simulink model "commhdlQPSKTxRx"  (R2025b)
settings: Solver=FixedStepDiscrete  StartTime=0.0  StopTime=stopTime  RelTol=1e-3
PostLoadFcn:
  | hScopeConfig = get_param([gcs '/Receiver/QPSK Rx/Frequency and Time Synchronizer/Symbol Synchronizer/No HDL/QPSK Receiver Eye Diagram'],'ScopeConfiguration');
  | 
  | hScopeConfig.OpenAtSimulationStart = false;
  | hScopeConfig.Visible = false;
  | SamplesPerSymbol = 4;
  | %UpsamplesRx = 1;
  | clear hScopeConfig
InitFcn:
  | commhdlQPSKTxRxModelInit;
  | % Rate bridge: ADRV9002/Jupiter radio runs at 15.36 MHz = 2x the 7.68 MHz
  | % (4 samples/symbol @ Rsym=1.92 MHz) the QPSK Rx requires. The deployed
  | % Receiver must downsample the ADC stream by 2. UpsamplesRx=1 fed the QPSK
  | % Rx 8 sps (2x-upsampled) and broke symbol sync / the loopback bit check.
  | UpsamplesRx = 1;   %% T8 RATE FIX: rail 15.36e6 == ADC bus rate,
  | %% no ingress decimation (was 2 when the rail sat on the 7.68e6 rung)
  | UpsamplesTx = 1;
  | clear simTimingOffset;
StopFcn:
  | if exist('simTimingOffset','var')
  |   disp('Simulation completed');
  |   %QPSKTxRxVerification;
  | end
undefined symbols (not defined in the file or in its folder): Add, Config, fsym, randsrc, RandStream, Rsym, Shift
libraries: hdlsllib x76, simulink x21, dspsigops x19, dsphdlfiltering2 x3, dsphdlsigops2 x2, dsphdlmathfun2 x2, commdigbbndpm3 x2, commchan3 x1, commrflib2 x1
(part 4 of 4)

== matlab function commhdlQPSKTxRx/Receiver/QPSK Rx/Frequency and Time Synchronizer/Packet Controller/sample discard controller ==
  data: dataIn input; validIn input; dataOut output; startIn input; endIn input; startOut output; endOut output; validOut output
function [dataOut,startOut,endOut,validOut] = controller(dataIn,validIn,startIn,endIn)
%#codegen

   persistent active dataOutReg validOutReg startOutReg endOutReg;
   if isempty(active)
      active  = false;
      dataOutReg = cast(0,'like',dataIn);
      validOutReg = false;
      startOutReg = false;
      endOutReg = false;
   end
   
   dataOut = dataOutReg;
   validOut = validOutReg;
   startOut = startOutReg;
   endOut = endOutReg;
   
   startOutReg = startIn;
   endOutReg = endIn;
   
   if startIn
       active = true;
   end
   
   if active
       dataOutReg(:) = dataIn;
       validOutReg = validIn;
   else
       dataOutReg(:) = 0;
       validOutReg = false;
   end
   
   if endIn
       if active 
           endOutReg = true;
       else
           endOutReg = false;
       end
       active = false;
   end
end

== matlab function commhdlQPSKTxRx/Receiver/QPSK Rx/Frequency and Time Synchronizer/Symbol Synchronizer/Interpolation Control ==
  data: mu output; Delta input; Underflow output
function [mu,Underflow] = Interpolation_ctrl(Delta)
% Implementation of modulo-1 counter for interpolation control listed in
% Figure 8.4.19 of "Digital Communications - A Discrete-Time Approach"
% by Michael Rice. See design details in Chapter 8.4.3 of the same book.
% 
% Input:
%   Delta - Loop filter output. If loop is in lock, delta would be small
% Output:
%   Underflow - Indicator of counter underflow. This is the strobe signal
%               for downstream processing
%   mu - Difference between actual sampling instant and the optimal instant,
%        between zero and one
%#codegen

% countReg - Counter value delayed by 1 sample
% muReg - The estimated timing error normalized by half QPSK symbols

   mask = fi(1-2^(-10),1,11,10);
   
   persistent countReg underflowReg muReg;
   if isempty(countReg)
       countReg  = fi(0,1,11,10);
       muReg = fi(0,1,11,10);
       underflowReg = false;
   end
   
   
   Underflow = underflowReg;
   mu = muReg;   
   
   
      % T8.4 anti-wedge clamp: if Delta <= -0.125 the decrementing counter
   % never underflows (strobes stop FOREVER -- Class-4 wedge / Class-1
   % episode mechanism; see tb_timing_wedge.v). Bound Delta so the
   % counter always decrements by >= 1 LSB.
   wlim = fi(255/1024,1,11,10);
   if Delta > wlim
       Delta = wlim;
   elseif Delta < -wlim
       Delta = fi(-255/1024,1,11,10);
   end
   counter = bitand(mask,countReg)-Delta-fi(0.25,1,11,10); % decrementing counter
   
   % if countReg is a nonnegative number,
   % then mod(countReg,1) equals the fractional part of countReg
   if counter < 0
       underflowReg = true;
       muReg = bitshift(bitand(mask,countReg),2);
       countReg = fi(counter+1,1,11,10);% create underflow to counter
   else
       underflowReg = false;
       countReg = fi(counter,1,11,10);
   end
   


end

== matlab function commhdlQPSKTxRx/Receiver/QPSK Rx/Frequency and Time Synchronizer/Preamble Detector/Correlator/ThresholdLimiter ==
  settings: fimath=hdlfimath
  data: x input; y output
function y = applyLowerLimit(x)
    % Apply a lower limit to the threshold.
    %#codegen
    
    % Threshold is computed by summing across 63 samples.
    % Set lower limit to be equivalent of all 63 samples
    % having their LSB set to 1 and all others set to 0. 
    lowerLimit = cast(0.01, 'like', x);
    
    if x < lowerLimit
        y = lowerLimit;
    else
        y = x;
    end
end

== matlab function commhdlQPSKTxRx/Transmitter/Input Data/Message Generator/MATLAB Function ==
  data: enable input; reset input; out output; start output; stop output; valid output; count_out output; msg_count_out output
function [out, start, stop, valid, count_out, msg_count_out] = msggen(enable, reset)

persistent indexCount;
persistent toggle;
persistent msgCount;
persistent msgCountAll;
persistent msgCountBitIndex;

if isempty(indexCount) || isempty(toggle) || isempty(msgCount) || isempty(msgCountBitIndex) || isempty(msgCountAll)
    indexCount = uint32(0);
    msgCount = uint32(1);
    msgCountAll = uint32(1);
    msgCountBitIndex = uint8(0);
    toggle = false;
end

%% Constants
strAscii = dec2bin('ADI Hello World', 8);
msgarray = reshape(strAscii', [1, numel(strAscii)]);
msgbits = logical(msgarray - 48);
msgbitsLen = length(msgbits);

fullMessageLen = uint32(2240-1); % Need the -1 to eat the feedback delay

% Bit counter
% N = 8;% 8-bit counter
% mask = uint32(2^N - 1);
% for k = 1:300
%     msgCount = bitand(msgCount + uint32(1), mask);   % wraps 255 -> 0
% end

%% Logic
if enable && ~reset
    % Set out data
    if indexCount < msgbitsLen % Insert msg
        out = msgbits(indexCount + 1);
        msgCountBitIndex = uint8(0);
    else % Zero padding: varying filler (counter digit + toggle bits)
        % caused periodic false-lock error bursts in the deployed BIST;
        % zero-padded payload matches the verified host golden structure.
        out = false;
        msgCountBitIndex = uint8(0);
    end

    % Flags
    start = indexCount == uint32(0);
    stop = indexCount == fullMessageLen;
    valid = true;

    % Counters
    if fullMessageLen == indexCount
        if msgCount >= 9
            msgCount = uint32(1);
        else
            msgCount = msgCount +  1;
            msgCountAll = msgCountAll + 1;
        end
    end
    if indexCount <= fullMessageLen
        indexCount = indexCount + 1;
    end

else % Enable == false

    if reset
        indexCount = uint32(0);
        % msgCount = uint32(0);
        msgCountBitIndex = uint8(0);
        toggle = false;
    end
    out = false;
    start = false;
    stop = false;
    valid = false;
end

if isempty(indexCount)
    count_out = uint32(0);
else
    count_out = indexCount;
end

msg_count_out = msgCountAll;

== matlab function commhdlQPSKTxRx/Receiver/QPSK Rx/Frequency and Time Synchronizer/Symbol Synchronizer/Rate Handle/FIFO/Validate Input Push Pop/No HDL/MATLAB Function ==
  data: pushFullDiag input; popEmptyDiag input; pushFull input; popEmpty input
function pushPopDiagnostics(pushFullDiag, popEmptyDiag, pushFull, popEmpty)
%#codegen


if(pushFull)
    switch pushFullDiag
        case 2
            warning('Push signal applied on full FIFO');
        case 3
            error('Push signal applied on full FIFO');
        otherwise
    end
end

if(popEmpty)
    switch popEmptyDiag
        case 2
            warning('Pop signal applied on empty FIFO');
        case 3
            error('Pop signal applied on empty FIFO');
        otherwise
    end
end

end
